simulink model "Model"  (R2024b)
settings: Solver=VariableStepAuto  StartTime=0.0  StopTime=12  RelTol=1e-4
values from neighbouring files (symbols this model uses):
  s = tf('s')    [inspect_bandwidth.m]
undefined symbols (not defined in the file or in its folder): G1, Joint1, kontrolculer, L1, M1, X, Y, Z
libraries: sm_lib x6, slpidlib x3, nesl_utility x2, simulink x1
settings Model: Creator=msaidd  LastModifiedBy=AnEng

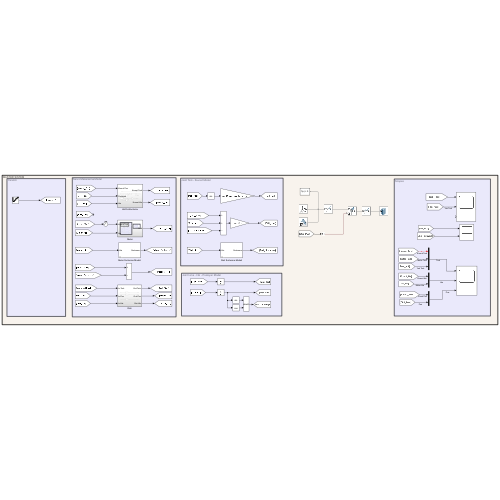
[thumbnail: Simulink's stored preview of the top-level diagram]
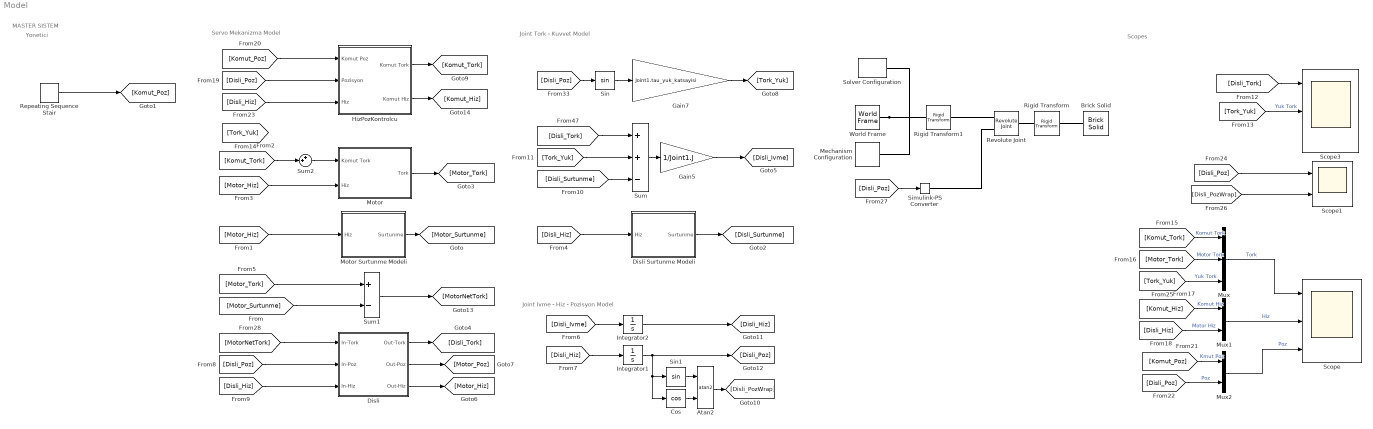
== system Model ==
  note: Yonetici
  note: Joint Ivme - Hiz - Pozisyon Model
  note: Servo Mekanizma Model
  note: MASTER SISTEM
  note: Scopes
  note: Joint Tork - Kuvvet Model
  Atan2 : Trigonometry  Operator=atan2
  Brick Solid : sm_lib/Body Elements/Brick Solid  BrickDimensions=[L1.width L1.thickness L1.length]  BrickDimensionsUnits=m  ExportEntireGeometry=off  InertiaType=CalculateFromGeometry  BasedOnType=Density  Density=L1.rho  DensityUnits=kg/m^3  Mass=1  MassUnits=kg  CenterOfMass=[0 0 0]  CenterOfMassUnits=m  MomentsOfInertia=[1 1 1]  MomentsOfInertiaUnits=kg*m^2  ProductsOfInertia=[0 0 0]  ProductsOfInertiaUnits=kg*m^2  GraphicType=FromGeometry  MarkerShape=Sphere  MarkerSize=10  GraphicVisPropType=SimpleVisualProperties  GraphicDiffuseColor=[0.5 0.5 0.5]  GraphicOpacity=1  GraphicSpecularColor=[0.5 0.5 0.5 1.0]  GraphicAmbientColor=[0.15 0.15 0.15 1.0]  GraphicEmissiveColor=[0.0 0.0 0.0 1.0]  GraphicShininess=75  DoExposeReferenceFrame=on  SerializedFrames=<Frames/>
  Cos : Trigonometry  Operator=cos
  Disli : Subsystem
  Disli Surtunme Modeli : Subsystem  mask{P=G1}
      mask prompts: P "Surtunme Struct"
  Gain5 : Gain  Gain=1/Joint1.J
  Gain7 : Gain  Gain=Joint1.tau_yuk_katsayisi
  HizPozKontrolcu : Subsystem
  Integrator1 : Integrator
  Integrator2 : Integrator
  Mechanism Configuration : sm_lib/Utilities/Mechanism Configuration  UniformGravity=Constant  GravityVector=[0 0 -9.81]  GravityVectorUnits=m/s^2  LinearizationDelta=0.001  JointModeTransitionNonlinearIterations=2
  Motor : Subsystem
  Motor Surtunme Modeli : Subsystem  mask{P=M1}
      mask prompts: P "Surtunme Struct"
  Mux : Mux  Inputs=3
  Mux1 : Mux  Inputs=2
  Mux2 : Mux  Inputs=2
  Repeating Sequence Stair : simulink/Sources/Repeating Sequence Stair  OutValues=[pi/2 pi 3*pi/2 2*pi].'  tsamp=3  OutMin=[]  OutMax=[]  OutDataTypeStr=double  OutputDataTypeScalingMode=double  OutDataType=fixdt(0,8)  ConRadixGroup=Best Precision: Vector-wise  OutScaling=2^-12
  Revolute Joint : sm_lib/Joints/Revolute Joint  JointMode=Normal  CompositeWrenchDir=FollowerOnBase  CompositeWrenchFrame=BaseFrame  SenseConstraintForce=off  SenseConstraintTorque=off  SenseTotalForce=off  SenseTotalTorque=off  PositionTargetSpecify=off  PositionTargetPriority=High  PositionTargetValue=0  PositionTargetValueUnits=deg  VelocityTargetSpecify=off  VelocityTargetPriority=High  VelocityTargetValue=0  VelocityTargetValueUnits=deg/s  EquilibriumPosition=0  EquilibriumPositionUnits=deg  SpringStiffness=0  SpringStiffnessUnits=N*m/deg  DampingCoefficient=0  DampingCoefficientUnits=N*m/(deg/s)  LowerLimitSpecify=off  LowerLimitBound=-90  LowerLimitBoundUnits=deg  LowerLimitStiffness=1e4  LowerLimitStiffnessUnits=N*m/deg  LowerLimitDamping=10  LowerLimitDampingUnits=N*m/(deg/s)  LowerLimitTransitionRegionWidth=0.1  LowerLimitTransitionRegionWidthUnits=deg  UpperLimitSpecify=off  UpperLimitBound=90  UpperLimitBoundUnits=deg  UpperLimitStiffness=1e4  UpperLimitStiffnessUnits=N*m/deg  UpperLimitDamping=10  UpperLimitDampingUnits=N*m/(deg/s)  UpperLimitTransitionRegionWidth=0.1  UpperLimitTransitionRegionWidthUnits=deg  TorqueActuationMode=ComputedTorque  MotionActuationMode=InputMotion  SensePosition=off  SenseVelocity=off  SenseAcceleration=off  SenseTorqueForce=off  SenseLowerLimitTorqueForce=off  SenseUpperLimitTorqueForce=off
  Rigid Transform : sm_lib/Frames and Transforms/Rigid Transform  RotationMethod=StandardAxis  FollAlignAxisA=+X  BaseAlignAxisA=+Y  FollAlignAxisB=+Y  BaseAlignAxisB=+Z  RotationStandardAxis=+X  RotationAngle=-90  RotationAngleUnits=deg  RotationArbitraryAxis=[0 0 1]  RotationSequenceAxes=FollowerAxes  RotationSequence=XYX  RotationSequenceAngles=[0 0 0]  RotationSequenceAnglesUnits=deg  RotationMatrix=[1 0 0;0 1 0;0 0 1]  Quaternion=[1 0 0 0]  TranslationMethod=StandardAxis  TranslationCartesianOffset=[0 0 0]  TranslationCartesianOffsetUnits=m  TranslationStandardAxis=+Y  TranslationStandardOffset=L1.lc  TranslationStandardOffsetUnits=m  TranslationROffset=0  TranslationROffsetUnits=m  TranslationThetaOffset=0  TranslationThetaOffsetUnits=deg  TranslationZOffset=0  TranslationZOffsetUnits=m
  Rigid Transform1 : sm_lib/Frames and Transforms/Rigid Transform  RotationMethod=StandardAxis  FollAlignAxisA=+X  BaseAlignAxisA=+Y  FollAlignAxisB=+Y  BaseAlignAxisB=+Z  RotationStandardAxis=+X  RotationAngle=90  RotationAngleUnits=deg  RotationArbitraryAxis=[0 0 1]  RotationSequenceAxes=FollowerAxes  RotationSequence=XYX  RotationSequenceAngles=[0 0 0]  RotationSequenceAnglesUnits=deg  RotationMatrix=[1 0 0;0 1 0;0 0 1]  Quaternion=[1 0 0 0]  TranslationMethod=None  TranslationCartesianOffset=[0 0 0]  TranslationCartesianOffsetUnits=m  TranslationStandardAxis=+Y  TranslationStandardOffset=L1.lc  TranslationStandardOffsetUnits=m  TranslationROffset=0  TranslationROffsetUnits=m  TranslationThetaOffset=0  TranslationThetaOffsetUnits=deg  TranslationZOffset=0  TranslationZOffsetUnits=m
  Scope : Scope  NumInputPorts=3
  Scope1 : Scope  NumInputPorts=2
  Scope3 : Scope  NumInputPorts=3
  Simulink-PS Converter : nesl_utility/Simulink-PS Converter  PhysicalDomain=network_engine_domain  SubClassName=ps_input  LeftPortType=input  RightPortType=output  PseudoPeriodic=off  Frequencies=[]  NoiseDistribution=none  NoiseParameters=[]  Unit=rad  AffineConversion=off  FilteringAndDerivatives=filter  SimscapeFilterOrder=2  InputFilterTimeConstant=0.001  UdotUserProvided=0
  Sin : Trigonometry
  Sin1 : Trigonometry
  Solver Configuration : nesl_utility/Solver Configuration  PhysicalDomain=network_engine_domain  SubClassName=solver  LeftPortType=input  RightPortType=generic  Tones=[]  Harmonics=[]  SimulateNoise=off  Profile=off  UseLocalSampling=off  EnableSwitchedLinearOptims=on  FrequencyDomain=off  UseCCode=off  RelTol=0.001  AbsTol=0.001  MinStep=1e-09  ToWorkspace=off  RevertToSquareIcSolve=off  NumHomotopyIterations=100  PhasorMode=off  PhasorModeNumHarmonics=1  ConsistencySolver=NEWTON_XTOL_AFTER_FTOL  IndexReductionMethod=DerivativeReplacement  DoDC=off  ResidualTolerance=1e-09  ConsistencyTolSource=GLOBAL  ConsistencyAbsTol=0.001  ConsistencyRelTol=0.001  ConsistencyTolFactor=0.001  UseLocalSolver=off  LocalSolverChoice=NE_BACKWARD_EULER_ADVANCER  ResolveIndetEquations=on  FunctionEvalNumThread=1  LocalSolverSampleTime=0.001  DoFixedCost=off  MaxNonlinIter=3  MaxModeIter=2  ComputeImpulses=off  ImpulseIterations=2  LinearAlgebra=auto  LinearAlgebraNumThread=0  EquationFormulation=NE_TIME_EF  DelaysMemoryBudget=1024  AutomaticFiltering=on  FilteringTimeConstant=0.001  PartitionStorageMethod=AS_NEEDED  PartitionMemoryBudget=1024  PartitionMethod=ROBUST  MultibodyUseLocalSolver=off  MultibodyLocalSolverChoice=ODE1  MultibodyLocalSolverSampleTime=0.001
  Sum : Sum  Inputs=++-
  Sum1 : Sum  Inputs=+-
  Sum2 : Sum  Inputs=++|
  World Frame : sm_lib/Frames and Transforms/World Frame
  wires:
  [Disli_Poz] -> Sin/1
  Sin/1 -> Gain7/1
  Gain7/1 -> [Tork_Yuk]
  Gain5/1 -> [Disli_Ivme]
  [Tork_Yuk] -> Sum/2
  [Disli_Tork] -> Sum/1
  Sum/1 -> Gain5/1
  [Motor_Hiz] -> Motor/2(Hiz)
  Motor/1(Tork) -> [Motor_Tork]
  Disli/1(Out-Tork) -> [Disli_Tork]
  Disli Surtunme Modeli/1(Surtunme) -> [Disli_Surtunme]
  [Disli_Ivme] -> Integrator2/1
  Integrator2/1 -> [Disli_Hiz]
  [Motor_Tork] -> Sum1/1
  [Motor_Surtunme] -> Sum1/2
  [Disli_Hiz] -> Disli Surtunme Modeli/1(Hiz)
  [Disli_Surtunme] -> Sum/3
  [Disli_Tork] -> Scope3/1
  Mux/1 -> Scope/1  "Tork"
  [Komut_Tork] -> Mux/1  "Komut Tork"
  [Motor_Tork] -> Mux/2  "Motor Tork"
  [Disli_Hiz] -> Mux1/2  "Motor Hiz"
  [Komut_Hiz] -> Mux1/1  "Komut Hiz"
  Mux1/1 -> Scope/2  "Hiz"
  Mux2/1 -> Scope/3  "Poz"
  [Disli_Poz] -> Mux2/2  "Poz"
  [Komut_Poz] -> Mux2/1  "Kmut Poz"
  [Tork_Yuk] -> Mux/3  "Yuk Tork"
  HizPozKontrolcu/1(Komut Tork) -> [Komut_Tork]
  [Disli_Poz] -> HizPozKontrolcu/2(Pozisyon)
  [Disli_Hiz] -> HizPozKontrolcu/3(Hiz)
  [Komut_Tork] -> Sum2/2
  Sum2/1 -> Motor/1(Komut Tork)
  [Tork_Yuk] -> Scope3/2  "Yuk Tork"
  [Komut_Poz] -> HizPozKontrolcu/1(Komut Poz)
  HizPozKontrolcu/2(Komut Hiz) -> [Komut_Hiz]
  [Disli_Hiz] -> Integrator1/1
  [Disli_Poz] -> Scope1/1
  [Disli_PozWrap] -> Scope1/2
  Integrator1/1 -> Cos/1, Sin1/1, [Disli_Poz]
  Atan2/1 -> [Disli_PozWrap]
  Sin1/1 -> Atan2/1
  Cos/1 -> Atan2/2
  Repeating Sequence Stair/1 -> [Komut_Poz]
  [Disli_Poz] -> Simulink-PS Converter/1
  Disli/2(Out-Poz) -> [Motor_Poz]
  Disli/3(Out-Hiz) -> [Motor_Hiz]
  [Disli_Poz] -> Disli/2(In-Poz)
  [Disli_Hiz] -> Disli/3(In-Hiz)
  Sum1/1 -> [MotorNetTork]
  Motor Surtunme Modeli/1(Surtunme) -> [Motor_Surtunme]
  [Motor_Hiz] -> Motor Surtunme Modeli/1(Hiz)
  [MotorNetTork] -> Disli/1(In-Tork)
  connections:
  World Frame/RConn1 -- Rigid Transform1/LConn1 -- Mechanism Configuration/RConn1 -- Solver Configuration/RConn1
  Brick Solid/RConn1 -- Rigid Transform/RConn1
  Rigid Transform/LConn1 -- Revolute Joint/RConn1
  Revolute Joint/LConn2 -- Simulink-PS Converter/RConn1
  Rigid Transform1/RConn1 -- Revolute Joint/LConn1

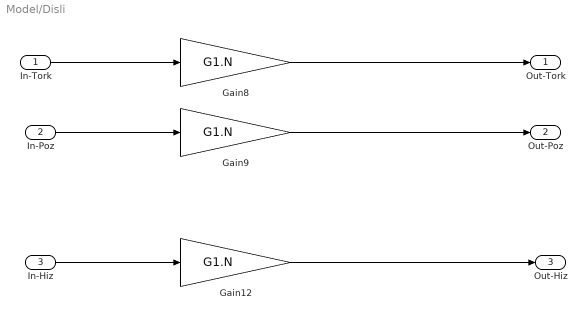
== system Model/Disli ==
  In-Tork : Inport
  In-Poz : Inport  Port=2
  In-Hiz : Inport  Port=3
  Gain12 : Gain  Gain=G1.N
  Gain8 : Gain  Gain=G1.N
  Gain9 : Gain  Gain=G1.N
  Out-Tork : Outport
  Out-Poz : Outport  Port=2
  Out-Hiz : Outport  Port=3
  wires:
  In-Tork/1 -> Gain8/1
  Gain9/1 -> Out-Poz/1
  In-Poz/1 -> Gain9/1
  In-Hiz/1 -> Gain12/1
  Gain12/1 -> Out-Hiz/1
  Gain8/1 -> Out-Tork/1

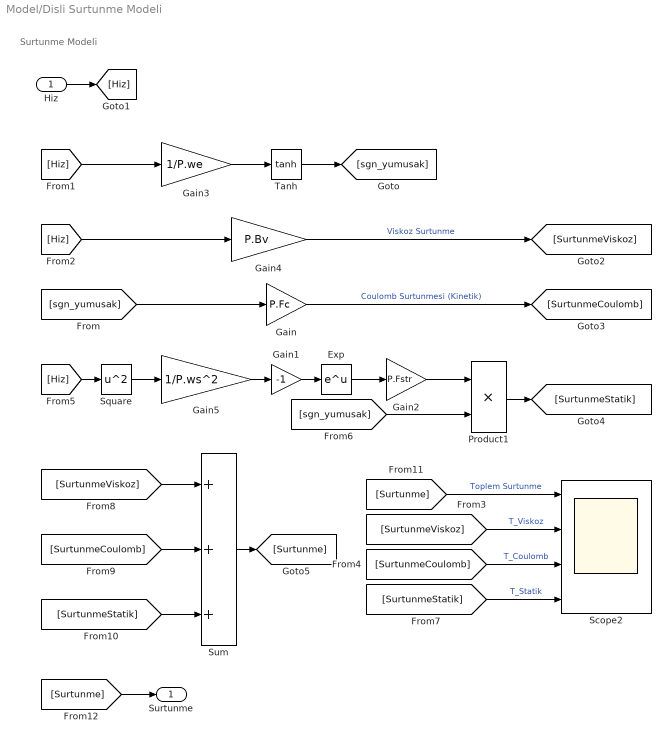
== system Model/Disli Surtunme Modeli ==
  note: Surtunme Modeli
  Hiz : Inport
  Exp : Math
  Gain : Gain  Gain=P.Fc
  Gain1 : Gain  Gain=-1
  Gain2 : Gain  Gain=P.Fstr
  Gain3 : Gain  Gain=1/P.we
  Gain4 : Gain  Gain=P.Bv
  Gain5 : Gain  Gain=1/P.ws^2
  Product1 : Product
  Scope2 : Scope  NumInputPorts=4
  Square : Math  Operator=square
  Sum : Sum  Inputs=+++
  Tanh : Trigonometry  Operator=tanh
  Surtunme : Outport
  wires:
  Gain4/1 -> [SurtunmeViskoz]  "Viskoz Surtunme"
  Gain/1 -> [SurtunmeCoulomb]  "Coulomb Surtunmesi (Kinetik)"
  [Hiz] -> Gain4/1
  Sum/1 -> [Surtunme]
  [SurtunmeViskoz] -> Scope2/2  "T_Viskoz"
  [SurtunmeCoulomb] -> Scope2/3  "T_Coulomb"
  [SurtunmeStatik] -> Scope2/4  "T_Statik"
  [Hiz] -> Gain3/1
  Gain3/1 -> Tanh/1
  Tanh/1 -> [sgn_yumusak]
  Hiz/1 -> [Hiz]
  [sgn_yumusak] -> Gain/1
  [Hiz] -> Square/1
  Square/1 -> Gain5/1
  Gain1/1 -> Exp/1
  Exp/1 -> Gain2/1
  Gain2/1 -> Product1/1
  [sgn_yumusak] -> Product1/2
  Product1/1 -> [SurtunmeStatik]
  [SurtunmeViskoz] -> Sum/1
  [SurtunmeCoulomb] -> Sum/2
  [SurtunmeStatik] -> Sum/3
  [Surtunme] -> Scope2/1  "Toplem Surtunme"
  [Surtunme] -> Surtunme/1
  Gain5/1 -> Gain1/1

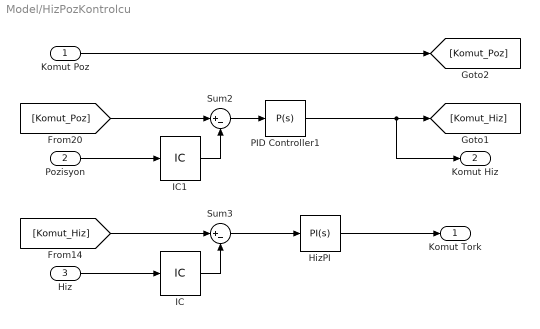
== system Model/HizPozKontrolcu ==
  Komut Poz : Inport
  Pozisyon : Inport  Port=2
  Hiz : Inport  Port=3
  HizPI : slpidlib/PID Controller  Controller=PI  Form=Ideal  TimeDomain=Continuous-time  UseExternalTs=off  SampleTime=-1  IntegratorMethod=Forward Euler  FilterMethod=Forward Euler  ControllerParametersSource=internal  P=kontrolculer.hiz.Kp  I=kontrolculer.hiz.Ki  UseKiTs=off  D=0  UseExternalDerivativeSource=off  N=100  UseFilter=on  TunerSelectOption=Transfer Function Based (PID Tuner App)  InitialConditionSource=internal  InitialConditionForIntegrator=0  InitialConditionForFilter=0  DifferentiatorICPrevScaledInput=0  ExternalReset=none  TrackingMode=off  Kt=1  LimitOutput=on  SatLimitsSource=internal  UpperSaturationLimit=0.0422  LowerSaturationLimit=-0.0422  LinearizeAsGain=on  AntiWindupMode=none  Kb=1  LimitIntegrator=off  UpperIntegratorSaturationLimit=inf  LowerIntegratorSaturationLimit=-inf  POutMin=[]  POutMax=[]  IOutMin=[]  IOutMax=[]  DOutMin=[]  DOutMax=[]  NOutMin=[]  NOutMax=[]  SumOutMin=[]  SumOutMax=[]  SaturationOutMin=[]  SaturationOutMax=[]  PParamMin=[]  PParamMax=[]  IParamMin=[]  IParamMax=[]  DParamMin=[]  DParamMax=[]  NParamMin=[]  NParamMax=[]  KbParamMin=[]  KbParamMax=[]  KtParamMin=[]  KtParamMax=[]  KbOutMin=[]  KbOutMax=[]  KtOutMin=[]  KtOutMax=[]  IntegratorOutMin=[]  IntegratorOutMax=[]  FilterOutMin=[]  FilterOutMax=[]  SumI1OutMin=[]  SumI1OutMax=[]  SumI2OutMin=[]  SumI2OutMax=[]  SumI3OutMin=[]  SumI3OutMax=[]  SumI4OutMin=[]  SumI4OutMax=[]  SumDOutMin=[]  SumDOutMax=[]  DifferentiatorOutMin=[]  DifferentiatorOutMax=[]  FilterDiffOutCoefMin=[]  FilterDiffOutCoefMax=[]  ReciprocalOutMin=[]  ReciprocalOutMax=[]  SumDenOutMin=[]  SumDenOutMax=[]  SumNumOutMin=[]  SumNumOutMax=[]  DivideOutMin=[]  DivideOutMax=[]  UdiffTsProdOutMin=[]  UdiffTsProdOutMax=[]  NTsProdOutMin=[]  NTsProdOutMax=[]  UintegralTsProdOutMin=[]  UintegralTsProdOutMax=[]  UngainTsProdOutMin=[]  UngainTsProdOutMax=[]  ClampingZeroOutDataTypeStr=Inherit: Inherit via back propagation  ClampingZeroOutMin=[]  ClampingZeroOutMax=[]  FilterDenConstantOutDataTypeStr=Inherit: Inherit via back propagation  FilterDenConstantOutMin=[]  FilterDenConstantOutMax=[]  PCopyOutDataTypeStr=Inherit: Inherit via back propagation  PCopyOutMin=[]  PCopyOutMax=[]  NCopyOutDataTypeStr=Inherit: Inherit via back propagation  NCopyOutMin=[]  NCopyOutMax=[]  IntegratorContinuousStateAttributes=''  IntegratorStateMustResolveToSignalObject=off  IntegratorRTWStateStorageClass=Auto  FilterContinuousStateAttributes=''  FilterStateMustResolveToSignalObject=off  FilterRTWStateStorageClass=Auto  ParallelPVariant=Passthrough  IdealPVariant=InternalParameters  IVariant=InternalParameters  DVariant=Disabled  IntegratorVariant=Continuous  SatVariant=Enabled  AWVariant=Passthrough  PCopyVariant=Disabled  TRVariant=Disabled  FdbkBlocksVariant=Forward  IdealPFdbkVariant=Disabled  SatFdbkVariant=Disabled  DerivativeFilterVariant=Disabled  NVariant=Disabled  NCopyVariant=Disabled_SignalSpec  FilterICVariant=Disabled  IntegratorICVariant=InternalICs  ExternalResetVariant=Disabled  TRSumVariant=Passthrough  SumFdbkVariant=Disabled  SumVariant=Sum_PI  TsampFilterVariant=InternalTs  TsampNgainVariant=Passthrough  TsampIntegralVariant=Disabled_SignalSpec  ExternalSaturationOutDataTypeStr=Inherit: Same as second input  DerivativeSourceVariant=Disabled  PreIntVariant=InternalPreInt
  IC : InitialCondition  Value=0
  IC1 : InitialCondition  Value=0
  PID Controller1 : slpidlib/PID Controller  Controller=P  Form=Ideal  TimeDomain=Continuous-time  UseExternalTs=off  SampleTime=-1  IntegratorMethod=Forward Euler  FilterMethod=Forward Euler  ControllerParametersSource=internal  P=kontrolculer.poz.Kp  I=kontrolculer.hiz.Ki  UseKiTs=off  D=0  UseExternalDerivativeSource=off  N=100  UseFilter=on  TunerSelectOption=Transfer Function Based (PID Tuner App)  InitialConditionSource=internal  InitialConditionForIntegrator=0  InitialConditionForFilter=0  DifferentiatorICPrevScaledInput=0  ExternalReset=none  TrackingMode=off  Kt=1  LimitOutput=on  SatLimitsSource=internal  UpperSaturationLimit=2  LowerSaturationLimit=-2  LinearizeAsGain=on  AntiWindupMode=none  Kb=1  LimitIntegrator=off  UpperIntegratorSaturationLimit=inf  LowerIntegratorSaturationLimit=-inf  POutMin=[]  POutMax=[]  IOutMin=[]  IOutMax=[]  DOutMin=[]  DOutMax=[]  NOutMin=[]  NOutMax=[]  SumOutMin=[]  SumOutMax=[]  SaturationOutMin=[]  SaturationOutMax=[]  PParamMin=[]  PParamMax=[]  IParamMin=[]  IParamMax=[]  DParamMin=[]  DParamMax=[]  NParamMin=[]  NParamMax=[]  KbParamMin=[]  KbParamMax=[]  KtParamMin=[]  KtParamMax=[]  KbOutMin=[]  KbOutMax=[]  KtOutMin=[]  KtOutMax=[]  IntegratorOutMin=[]  IntegratorOutMax=[]  FilterOutMin=[]  FilterOutMax=[]  SumI1OutMin=[]  SumI1OutMax=[]  SumI2OutMin=[]  SumI2OutMax=[]  SumI3OutMin=[]  SumI3OutMax=[]  SumI4OutMin=[]  SumI4OutMax=[]  SumDOutMin=[]  SumDOutMax=[]  DifferentiatorOutMin=[]  DifferentiatorOutMax=[]  FilterDiffOutCoefMin=[]  FilterDiffOutCoefMax=[]  ReciprocalOutMin=[]  ReciprocalOutMax=[]  SumDenOutMin=[]  SumDenOutMax=[]  SumNumOutMin=[]  SumNumOutMax=[]  DivideOutMin=[]  DivideOutMax=[]  UdiffTsProdOutMin=[]  UdiffTsProdOutMax=[]  NTsProdOutMin=[]  NTsProdOutMax=[]  UintegralTsProdOutMin=[]  UintegralTsProdOutMax=[]  UngainTsProdOutMin=[]  UngainTsProdOutMax=[]  ClampingZeroOutDataTypeStr=Inherit: Inherit via back propagation  ClampingZeroOutMin=[]  ClampingZeroOutMax=[]  FilterDenConstantOutDataTypeStr=Inherit: Inherit via back propagation  FilterDenConstantOutMin=[]  FilterDenConstantOutMax=[]  PCopyOutDataTypeStr=Inherit: Inherit via back propagation  PCopyOutMin=[]  PCopyOutMax=[]  NCopyOutDataTypeStr=Inherit: Inherit via back propagation  NCopyOutMin=[]  NCopyOutMax=[]  IntegratorContinuousStateAttributes=''  IntegratorStateMustResolveToSignalObject=off  IntegratorRTWStateStorageClass=Auto  FilterContinuousStateAttributes=''  FilterStateMustResolveToSignalObject=off  FilterRTWStateStorageClass=Auto  ParallelPVariant=InternalParameters  IdealPVariant=Disabled  IVariant=Disabled  DVariant=Disabled  IntegratorVariant=Disabled  SatVariant=Enabled  AWVariant=Disabled  PCopyVariant=Disabled  TRVariant=Disabled  FdbkBlocksVariant=Forward  IdealPFdbkVariant=Disabled  SatFdbkVariant=Disabled  DerivativeFilterVariant=Disabled  NVariant=Disabled  NCopyVariant=Disabled_SignalSpec  FilterICVariant=Disabled  IntegratorICVariant=Disabled  ExternalResetVariant=Disabled  TRSumVariant=Passthrough  SumFdbkVariant=Disabled  SumVariant=Passthrough_P  TsampFilterVariant=InternalTs  TsampNgainVariant=Passthrough  TsampIntegralVariant=Disabled_SignalSpec  ExternalSaturationOutDataTypeStr=Inherit: Same as second input  DerivativeSourceVariant=Disabled  PreIntVariant=InternalPreInt
  Sum2 : Sum  Inputs=|+-
  Sum3 : Sum  Inputs=|+-
  Komut Tork : Outport
  Komut Hiz : Outport  Port=2
  wires:
  [Komut_Hiz] -> Sum3/1
  [Komut_Poz] -> Sum2/1
  Sum3/1 -> HizPI/1
  IC/1 -> Sum3/2
  IC1/1 -> Sum2/2
  Sum2/1 -> PID Controller1/1
  HizPI/1 -> Komut Tork/1
  Hiz/1 -> IC/1
  Komut Poz/1 -> [Komut_Poz]
  Pozisyon/1 -> IC1/1
  PID Controller1/1 -> Komut Hiz/1, [Komut_Hiz]

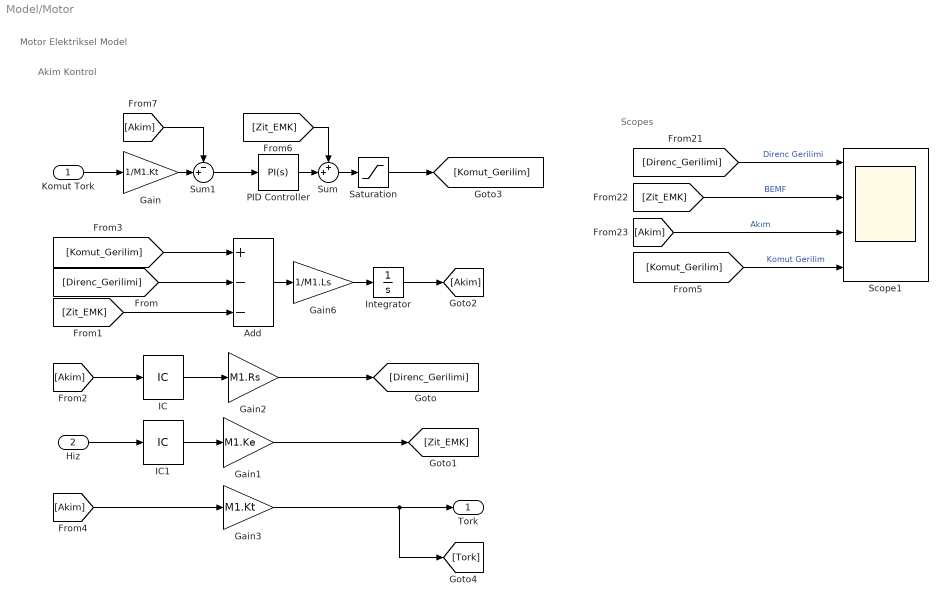
== system Model/Motor ==
  note: Scopes
  note: Motor Elektriksel Model
  note: Akim Kontrol
  Komut Tork : Inport
  Hiz : Inport  Port=2
  Add : Sum  Inputs=+--
  Gain : Gain  Gain=1/M1.Kt
  Gain1 : Gain  Gain=M1.Ke
  Gain2 : Gain  Gain=M1.Rs
  Gain3 : Gain  Gain=M1.Kt
  Gain6 : Gain  Gain=1/M1.Ls
  IC : InitialCondition  Value=0
  IC1 : InitialCondition  Value=0
  Integrator : Integrator
  PID Controller : slpidlib/PID Controller  Controller=PI  Form=Ideal  TimeDomain=Continuous-time  UseExternalTs=off  SampleTime=-1  IntegratorMethod=Forward Euler  FilterMethod=Forward Euler  ControllerParametersSource=internal  P=kontrolculer.akim.Kp  I=kontrolculer.akim.Ki  UseKiTs=off  D=0  UseExternalDerivativeSource=off  N=100  UseFilter=on  TunerSelectOption=Transfer Function Based (PID Tuner App)  InitialConditionSource=internal  InitialConditionForIntegrator=0  InitialConditionForFilter=0  DifferentiatorICPrevScaledInput=0  ExternalReset=none  TrackingMode=off  Kt=1  LimitOutput=on  SatLimitsSource=internal  UpperSaturationLimit=24  LowerSaturationLimit=-24  LinearizeAsGain=on  AntiWindupMode=back-calculation  Kb=kontrolculer.akim.Ki  LimitIntegrator=off  UpperIntegratorSaturationLimit=24  LowerIntegratorSaturationLimit=-24  POutMin=[]  POutMax=[]  IOutMin=[]  IOutMax=[]  DOutMin=[]  DOutMax=[]  NOutMin=[]  NOutMax=[]  SumOutMin=[]  SumOutMax=[]  SaturationOutMin=[]  SaturationOutMax=[]  PParamMin=[]  PParamMax=[]  IParamMin=[]  IParamMax=[]  DParamMin=[]  DParamMax=[]  NParamMin=[]  NParamMax=[]  KbParamMin=[]  KbParamMax=[]  KtParamMin=[]  KtParamMax=[]  KbOutMin=[]  KbOutMax=[]  KtOutMin=[]  KtOutMax=[]  IntegratorOutMin=[]  IntegratorOutMax=[]  FilterOutMin=[]  FilterOutMax=[]  SumI1OutMin=[]  SumI1OutMax=[]  SumI2OutMin=[]  SumI2OutMax=[]  SumI3OutMin=[]  SumI3OutMax=[]  SumI4OutMin=[]  SumI4OutMax=[]  SumDOutMin=[]  SumDOutMax=[]  DifferentiatorOutMin=[]  DifferentiatorOutMax=[]  FilterDiffOutCoefMin=[]  FilterDiffOutCoefMax=[]  ReciprocalOutMin=[]  ReciprocalOutMax=[]  SumDenOutMin=[]  SumDenOutMax=[]  SumNumOutMin=[]  SumNumOutMax=[]  DivideOutMin=[]  DivideOutMax=[]  UdiffTsProdOutMin=[]  UdiffTsProdOutMax=[]  NTsProdOutMin=[]  NTsProdOutMax=[]  UintegralTsProdOutMin=[]  UintegralTsProdOutMax=[]  UngainTsProdOutMin=[]  UngainTsProdOutMax=[]  ClampingZeroOutDataTypeStr=Inherit: Inherit via back propagation  ClampingZeroOutMin=[]  ClampingZeroOutMax=[]  FilterDenConstantOutDataTypeStr=Inherit: Inherit via back propagation  FilterDenConstantOutMin=[]  FilterDenConstantOutMax=[]  PCopyOutDataTypeStr=Inherit: Inherit via back propagation  PCopyOutMin=[]  PCopyOutMax=[]  NCopyOutDataTypeStr=Inherit: Inherit via back propagation  NCopyOutMin=[]  NCopyOutMax=[]  IntegratorContinuousStateAttributes=''  IntegratorStateMustResolveToSignalObject=off  IntegratorRTWStateStorageClass=Auto  FilterContinuousStateAttributes=''  FilterStateMustResolveToSignalObject=off  FilterRTWStateStorageClass=Auto  ParallelPVariant=Passthrough  IdealPVariant=InternalParameters  IVariant=InternalParameters  DVariant=Disabled  IntegratorVariant=Continuous  SatVariant=Enabled  AWVariant=BackCalculation  PCopyVariant=Disabled  TRVariant=Disabled  FdbkBlocksVariant=Forward  IdealPFdbkVariant=Disabled  SatFdbkVariant=Disabled  DerivativeFilterVariant=Disabled  NVariant=Disabled  NCopyVariant=Disabled_SignalSpec  FilterICVariant=Disabled  IntegratorICVariant=InternalICs  ExternalResetVariant=Disabled  TRSumVariant=Passthrough  SumFdbkVariant=Disabled  SumVariant=Sum_PI  TsampFilterVariant=InternalTs  TsampNgainVariant=Passthrough  TsampIntegralVariant=Disabled_SignalSpec  ExternalSaturationOutDataTypeStr=Inherit: Same as second input  DerivativeSourceVariant=Disabled  PreIntVariant=InternalPreInt
  Saturation : Saturate  UpperLimit=24  LowerLimit=-24
  Scope1 : Scope  NumInputPorts=4
  Sum : Sum  Inputs=++|
  Sum1 : Sum  Inputs=-+|
  Tork : Outport
  wires:
  Gain2/1 -> [Direnc_Gerilimi]
  [Zit_EMK] -> Add/3
  [Akim] -> Gain3/1
  [Akim] -> IC/1
  Integrator/1 -> [Akim]
  [Direnc_Gerilimi] -> Add/2
  Gain6/1 -> Integrator/1
  IC1/1 -> Gain1/1
  Gain1/1 -> [Zit_EMK]
  Add/1 -> Gain6/1
  IC/1 -> Gain2/1
  Gain3/1 -> [Tork], Tork/1
  Hiz/1 -> IC1/1
  [Komut_Gerilim] -> Add/1
  [Direnc_Gerilimi] -> Scope1/1  "Direnc Gerilimi"
  [Zit_EMK] -> Scope1/2  "BEMF"
  [Akim] -> Scope1/3  "Akım"
  [Komut_Gerilim] -> Scope1/4  "Komut Gerilim"
  Sum/1 -> Saturation/1
  [Zit_EMK] -> Sum/1
  Komut Tork/1 -> Gain/1
  PID Controller/1 -> Sum/2
  Saturation/1 -> [Komut_Gerilim]
  Gain/1 -> Sum1/2
  Sum1/1 -> PID Controller/1
  [Akim] -> Sum1/1

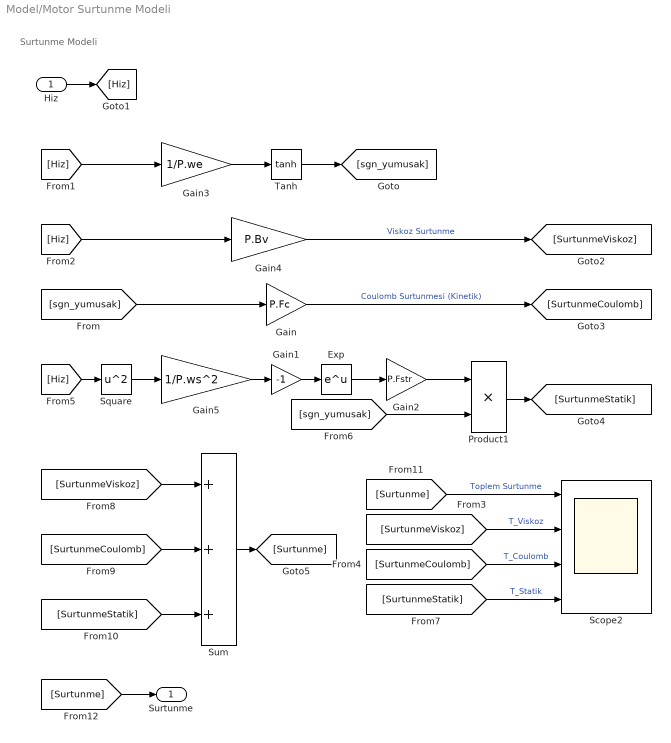
== system Model/Motor Surtunme Modeli ==
  note: Surtunme Modeli
  Hiz : Inport
  Exp : Math
  Gain : Gain  Gain=P.Fc
  Gain1 : Gain  Gain=-1
  Gain2 : Gain  Gain=P.Fstr
  Gain3 : Gain  Gain=1/P.we
  Gain4 : Gain  Gain=P.Bv
  Gain5 : Gain  Gain=1/P.ws^2
  Product1 : Product
  Scope2 : Scope  NumInputPorts=4
  Square : Math  Operator=square
  Sum : Sum  Inputs=+++
  Tanh : Trigonometry  Operator=tanh
  Surtunme : Outport
  wires:
  Gain4/1 -> [SurtunmeViskoz]  "Viskoz Surtunme"
  Gain/1 -> [SurtunmeCoulomb]  "Coulomb Surtunmesi (Kinetik)"
  [Hiz] -> Gain4/1
  Sum/1 -> [Surtunme]
  [SurtunmeViskoz] -> Scope2/2  "T_Viskoz"
  [SurtunmeCoulomb] -> Scope2/3  "T_Coulomb"
  [SurtunmeStatik] -> Scope2/4  "T_Statik"
  [Hiz] -> Gain3/1
  Gain3/1 -> Tanh/1
  Tanh/1 -> [sgn_yumusak]
  Hiz/1 -> [Hiz]
  [sgn_yumusak] -> Gain/1
  [Hiz] -> Square/1
  Square/1 -> Gain5/1
  Gain1/1 -> Exp/1
  Exp/1 -> Gain2/1
  Gain2/1 -> Product1/1
  [sgn_yumusak] -> Product1/2
  Product1/1 -> [SurtunmeStatik]
  [SurtunmeViskoz] -> Sum/1
  [SurtunmeCoulomb] -> Sum/2
  [SurtunmeStatik] -> Sum/3
  [Surtunme] -> Scope2/1  "Toplem Surtunme"
  [Surtunme] -> Surtunme/1
  Gain5/1 -> Gain1/1
